simulink model "Gr2_Ex5_2LinkRobot_FrictionEqGravity"  (R2024b)
settings: Solver=ode45  StartTime=0.0  StopTime=5  RelTol=1e-3
values from neighbouring files (symbols this model uses):
  dq0 = [0; 0]    [Gr2_Ex4_5_6_main.m]    (also in Gr2_Ex7_main.m; Gr2_Ex8_main.m)
  modelParameters = [m1, m2, l1, l2, g0, Fv]    [Gr2_Ex4_5_6_main.m]    (also in Gr2_Ex7_main.m = [m1 m2 l1 l2 g0 Fv]; Gr2_Ex8_main.m = [m1 m2 l1 l2 g0 Fv])
  q0 = [pi/2; pi/4]    [Gr2_Ex4_5_6_main.m]    (also in Gr2_Ex7_main.m = [0; pi/2]; Gr2_Ex8_main.m = [q1; q2])
settings Model: Creator=UX434  LastModifiedBy=UX434

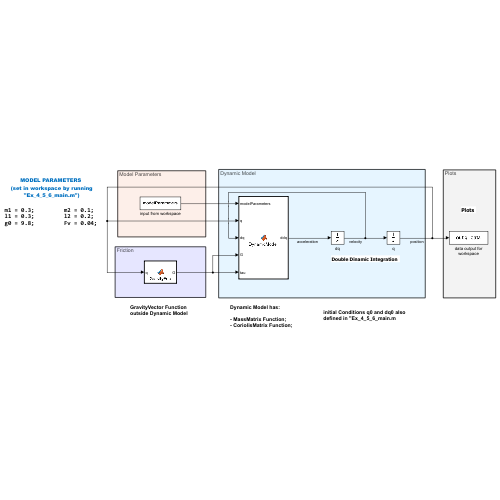
[thumbnail: Simulink's stored preview of the top-level diagram]
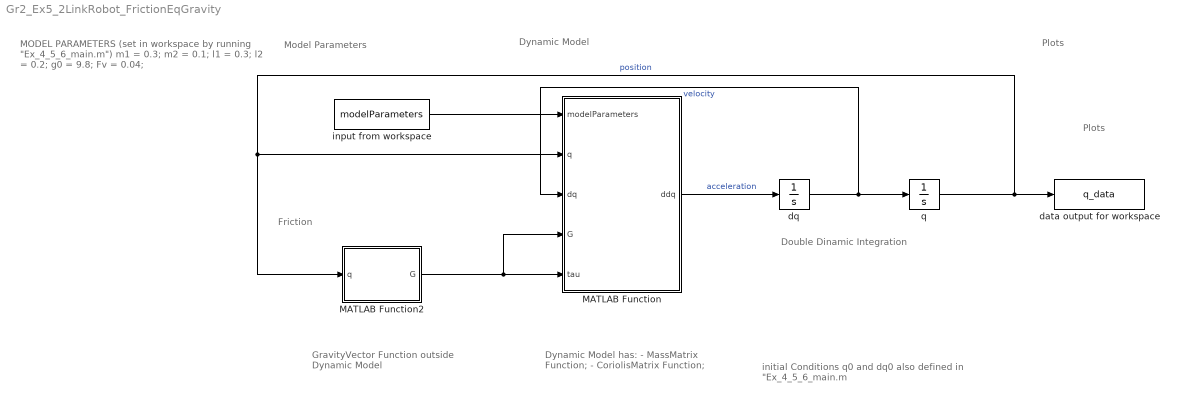
== system Gr2_Ex5_2LinkRobot_FrictionEqGravity ==
  note: Model Parameters
  note: Dynamic Model
  note: Friction
  note: Double Dinamic Integration
  note: Plots
  note: GravityVector Function outside Dynamic Model
  note: Dynamic Model has:
      |
      | - MassMatrix Function;
      | - CoriolisMatrix Function;
  note: Plots
  note: MODEL PARAMETERS
      | (set in workspace by running "Ex_4_5_6_main.m")
      |
      | m1 = 0.3; m2 = 0.1;
      | l1 = 0.3; l2 = 0.2;
      | g0 = 9.8; Fv = 0.04;
  note: initial Conditions q0 and dq0 also defined in "Ex_4_5_6_main.m
  MATLAB Function : MATLAB Function  TreatAsAtomicUnit=on
  MATLAB Function2 : MATLAB Function  TreatAsAtomicUnit=on
  data output for workspace : ToWorkspace  VariableName=q_data  SampleTime=-1
      settings: Save2DSignal=2-D array (concatenate along first dimension)
  dq : Integrator  InitialCondition=dq0
  input from workspace : Constant  Value=modelParameters
  q : Integrator  InitialCondition=q0
  wires:
  MATLAB Function/1(ddq) -> dq/1  "acceleration"
  dq/1 -> q/1, MATLAB Function/3(dq)  "velocity"
  q/1 -> data output for workspace/1, MATLAB Function2/1(q), MATLAB Function/2(q)  "position"
  MATLAB Function2/1(G) -> MATLAB Function/4(G), MATLAB Function/5(tau)
  input from workspace/1 -> MATLAB Function/1(modelParameters)

== matlab function Gr2_Ex5_2LinkRobot_FrictionEqGravity/MATLAB Function ==
  data: modelParameters input; ddq output; q input; dq input; G input; tau input
function ddq= DynamicModel(modelParameters, q, dq, G, tau)

m1 = modelParameters(1);         m2 = modelParameters(2); 
l1 = modelParameters(3);         l2 = modelParameters(4); 
g0 = modelParameters(5);         Fv = modelParameters(6);

lc1 = l1/2;  lc2 = l2/2;
I1czz = m1*l1^2/12;  I2czz = m2*l2^2/12;

M = Gr2_Ex3_MassMatrix(q, m1, m2, l1, lc1, lc2, I1czz, I2czz);
C = Gr2_Ex3_CoriolisMatrix(q, dq, m2, l1, lc2);

ddq = M \ (tau - C*dq - G - Fv*dq);

== matlab function Gr2_Ex5_2LinkRobot_FrictionEqGravity/MATLAB Function2 ==
  data: q input; G output
function G = GravityFnc(q)
m1 = 0.3;         m2 = 0.1; 
l1 = 0.3;         l2 = 0.2; 
g0 = 9.8;

lc1 = l1/2;  lc2 = l2/2; 

G = Gr2_Ex3_GravityVector(q, m1, m2, lc1, l1, lc2, g0);
